simulink model "AXU5EV_Hybrid_Reference_Check"  (R2026b)
settings: Solver=FixedStepDiscrete  StopTime=AX01B_Reference_Stop  FixedStep=Ts_ACR
undefined symbols (not defined in the file): Ts_ACR
settings Model: Creator=lww  LastModifiedBy=lww

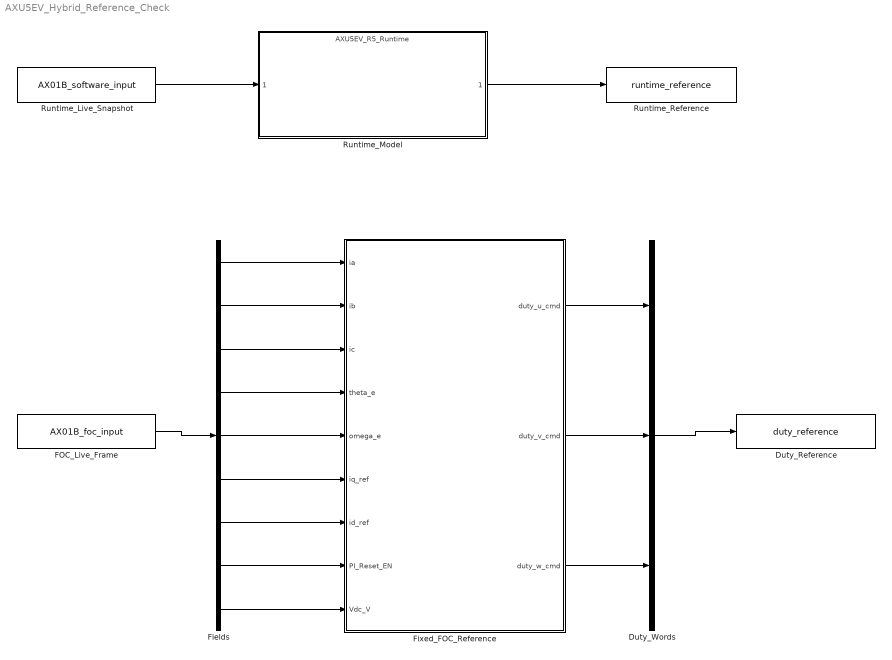
== system AXU5EV_Hybrid_Reference_Check ==
  Duty_Reference : ToWorkspace  VariableName=duty_reference  SaveFormat=Timeseries  SampleTime=-1
  Duty_Words : Mux  Inputs=3
  FOC_Live_Frame : FromWorkspace  VariableName=AX01B_foc_input  SampleTime=Ts_ACR  Interpolate=off  OutputAfterFinalValue=Holding final value
  Fields : Demux  Outputs=9
  Fixed_FOC_Reference : Subsystem  VariantControl=FOC_Impl_Select == 1
  Runtime_Live_Snapshot : FromWorkspace  VariableName=AX01B_software_input  SampleTime=Ts_ACR  Interpolate=off  OutputAfterFinalValue=Holding final value
  Runtime_Model : ModelReference  ModelNameDialog=AXU5EV_R5_Runtime  SimulationMode=Normal  ModelReferenceVersion=1.10
  Runtime_Reference : ToWorkspace  VariableName=runtime_reference  SaveFormat=Timeseries  SampleTime=-1
  wires:
  Runtime_Model/1 -> Runtime_Reference/1
  Runtime_Live_Snapshot/1 -> Runtime_Model/1
  Fixed_FOC_Reference/3(duty_w_cmd) -> Duty_Words/3
  Fixed_FOC_Reference/2(duty_v_cmd) -> Duty_Words/2
  Fixed_FOC_Reference/1(duty_u_cmd) -> Duty_Words/1
  Fields/9 -> Fixed_FOC_Reference/9(Vdc_V)
  Fields/8 -> Fixed_FOC_Reference/8(PI_Reset_EN)
  Fields/7 -> Fixed_FOC_Reference/7(id_ref)
  Fields/6 -> Fixed_FOC_Reference/6(iq_ref)
  Fields/5 -> Fixed_FOC_Reference/5(omega_e)
  Fields/4 -> Fixed_FOC_Reference/4(theta_e)
  Fields/3 -> Fixed_FOC_Reference/3(ic)
  Fields/2 -> Fixed_FOC_Reference/2(ib)
  Fields/1 -> Fixed_FOC_Reference/1(ia)
  FOC_Live_Frame/1 -> Fields/1
  Duty_Words/1 -> Duty_Reference/1

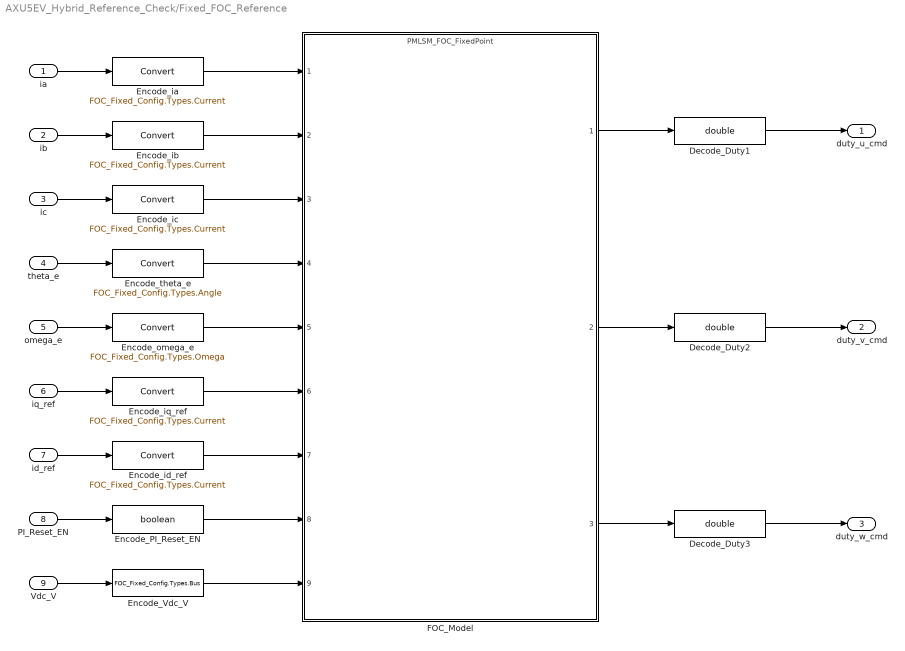
== system AXU5EV_Hybrid_Reference_Check/Fixed_FOC_Reference ==
  ia : Inport
  ib : Inport  Port=2
  ic : Inport  Port=3
  theta_e : Inport  Port=4
  omega_e : Inport  Port=5
  iq_ref : Inport  Port=6
  id_ref : Inport  Port=7
  PI_Reset_EN : Inport  Port=8
  Vdc_V : Inport  Port=9
  Decode_Duty1 : DataTypeConversion  OutDataTypeStr=double
  Decode_Duty2 : DataTypeConversion  OutDataTypeStr=double
  Decode_Duty3 : DataTypeConversion  OutDataTypeStr=double
  Encode_PI_Reset_EN : DataTypeConversion  OutDataTypeStr=boolean  RndMeth=Convergent
  Encode_Vdc_V : DataTypeConversion  OutDataTypeStr=FOC_Fixed_Config.Types.Bus  RndMeth=Convergent
  Encode_ia : DataTypeConversion  OutDataTypeStr=FOC_Fixed_Config.Types.Current  RndMeth=Convergent
  Encode_ib : DataTypeConversion  OutDataTypeStr=FOC_Fixed_Config.Types.Current  RndMeth=Convergent
  Encode_ic : DataTypeConversion  OutDataTypeStr=FOC_Fixed_Config.Types.Current  RndMeth=Convergent
  Encode_id_ref : DataTypeConversion  OutDataTypeStr=FOC_Fixed_Config.Types.Current  RndMeth=Convergent
  Encode_iq_ref : DataTypeConversion  OutDataTypeStr=FOC_Fixed_Config.Types.Current  RndMeth=Convergent
  Encode_omega_e : DataTypeConversion  OutDataTypeStr=FOC_Fixed_Config.Types.Omega  RndMeth=Convergent
  Encode_theta_e : DataTypeConversion  OutDataTypeStr=FOC_Fixed_Config.Types.Angle  RndMeth=Convergent
  FOC_Model : ModelReference  ModelNameDialog=PMLSM_FOC_FixedPoint  SimulationMode=Normal  ModelReferenceVersion=1.16
  duty_u_cmd : Outport
  duty_v_cmd : Outport  Port=2
  duty_w_cmd : Outport  Port=3
  wires:
  Decode_Duty1/1 -> duty_u_cmd/1
  Decode_Duty2/1 -> duty_v_cmd/1
  Decode_Duty3/1 -> duty_w_cmd/1
  FOC_Model/3 -> Decode_Duty3/1
  FOC_Model/2 -> Decode_Duty2/1
  FOC_Model/1 -> Decode_Duty1/1
  Encode_Vdc_V/1 -> FOC_Model/9
  Encode_omega_e/1 -> FOC_Model/5
  Encode_iq_ref/1 -> FOC_Model/6
  Encode_id_ref/1 -> FOC_Model/7
  Encode_PI_Reset_EN/1 -> FOC_Model/8
  Encode_ib/1 -> FOC_Model/2
  Encode_ic/1 -> FOC_Model/3
  Encode_theta_e/1 -> FOC_Model/4
  Encode_ia/1 -> FOC_Model/1
  PI_Reset_EN/1 -> Encode_PI_Reset_EN/1
  id_ref/1 -> Encode_id_ref/1
  iq_ref/1 -> Encode_iq_ref/1
  Vdc_V/1 -> Encode_Vdc_V/1
  omega_e/1 -> Encode_omega_e/1
  theta_e/1 -> Encode_theta_e/1
  ic/1 -> Encode_ic/1
  ib/1 -> Encode_ib/1
  ia/1 -> Encode_ia/1
